simulink model "case30_governor"  (R2026a)
settings: Solver=ode14x  StopTime=8  FixedStep=0.001
values from neighbouring files (symbols this model uses):
  P = load('case30_simulink_data.mat')    [case30_build_model.m]    (also in case30_check_model.m = L.scenario_P(P0, B, Yr_pre, Vr_pre, TYPE, ALPHA, LOC, TF, TC; case30_compute_delta_p.m = P0; case30_compute_delta_p_small.m = P0; case30_generate_dataset.m = P0)
settings Model: Creator=rnoor  LastModifiedBy=rnoor

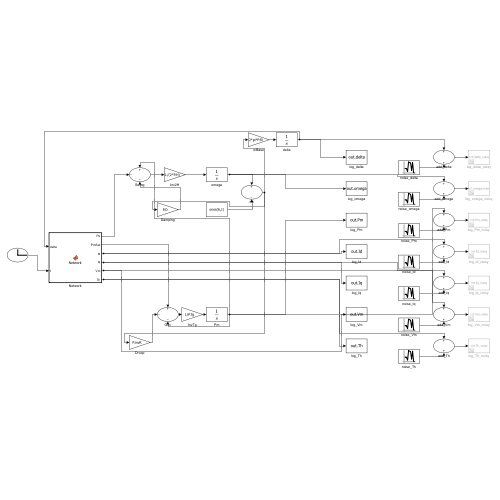
[thumbnail: Simulink's stored preview of the top-level diagram]
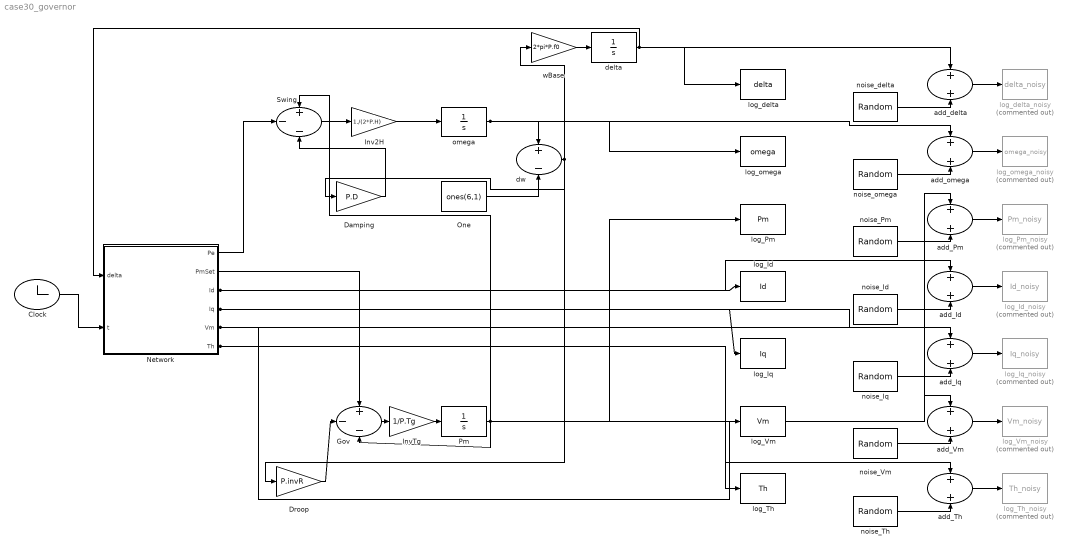
== system case30_governor ==
  Clock : Clock
  Damping : Gain  Gain=P.D
  Droop : Gain  Gain=P.invR
  Gov : Sum  Inputs=+--
  Inv2H : Gain  Gain=1./(2*P.H)
  InvTg : Gain  Gain=1/P.Tg
  Network : MATLAB Function  TreatAsAtomicUnit=on
  One : Constant  Value=ones(6,1)  VectorParams1D=off
  Pm : Integrator  InitialCondition=P.Pm0
  Swing : Sum  Inputs=+--
  add_Id : Sum
  add_Iq : Sum
  add_Pm : Sum
  add_Th : Sum
  add_Vm : Sum
  add_delta : Sum
  add_omega : Sum
  delta : Integrator  InitialCondition=P.delta0
  dw : Sum  Inputs=+-
  log_Id : ToWorkspace  VariableName=Id  SaveFormat=Timeseries  SampleTime=-1
  log_Id_noisy : ToWorkspace  Commented=on  VariableName=Id_noisy  SaveFormat=Timeseries  SampleTime=-1
  log_Iq : ToWorkspace  VariableName=Iq  SaveFormat=Timeseries  SampleTime=-1
  log_Iq_noisy : ToWorkspace  Commented=on  VariableName=Iq_noisy  SaveFormat=Timeseries  SampleTime=-1
  log_Pm : ToWorkspace  VariableName=Pm  SaveFormat=Timeseries  SampleTime=-1
  log_Pm_noisy : ToWorkspace  Commented=on  VariableName=Pm_noisy  SaveFormat=Timeseries  SampleTime=-1
  log_Th : ToWorkspace  VariableName=Th  SaveFormat=Timeseries  SampleTime=-1
  log_Th_noisy : ToWorkspace  Commented=on  VariableName=Th_noisy  SaveFormat=Timeseries  SampleTime=-1
  log_Vm : ToWorkspace  VariableName=Vm  SaveFormat=Timeseries  SampleTime=-1
  log_Vm_noisy : ToWorkspace  Commented=on  VariableName=Vm_noisy  SaveFormat=Timeseries  SampleTime=-1
  log_delta : ToWorkspace  VariableName=delta  SaveFormat=Timeseries  SampleTime=-1
  log_delta_noisy : ToWorkspace  Commented=on  VariableName=delta_noisy  SaveFormat=Timeseries  SampleTime=-1
  log_omega : ToWorkspace  VariableName=omega  SaveFormat=Timeseries  SampleTime=-1
  log_omega_noisy : ToWorkspace  Commented=on  VariableName=omega_noisy  SaveFormat=Timeseries  SampleTime=-1
  noise_Id : RandomNumber  Mean=zeros(6,1)  Variance=2.5e-05*ones(6,1)  Seed=400+(1:6)'  SampleTime=0.001  VectorParams1D=off
  noise_Iq : RandomNumber  Mean=zeros(6,1)  Variance=2.5e-05*ones(6,1)  Seed=500+(1:6)'  SampleTime=0.001  VectorParams1D=off
  noise_Pm : RandomNumber  Mean=zeros(6,1)  Variance=2.5e-05*ones(6,1)  Seed=300+(1:6)'  SampleTime=0.001  VectorParams1D=off
  noise_Th : RandomNumber  Mean=zeros(30,1)  Variance=0.0001*ones(30,1)  Seed=700+(1:30)'  SampleTime=0.001  VectorParams1D=off
  noise_Vm : RandomNumber  Mean=zeros(30,1)  Variance=1e-06*ones(30,1)  Seed=600+(1:30)'  SampleTime=0.001  VectorParams1D=off
  noise_delta : RandomNumber  Mean=zeros(6,1)  Variance=0.0001*ones(6,1)  Seed=100+(1:6)'  SampleTime=0.001  VectorParams1D=off
  noise_omega : RandomNumber  Mean=zeros(6,1)  Variance=2.5e-09*ones(6,1)  Seed=200+(1:6)'  SampleTime=0.001  VectorParams1D=off
  omega : Integrator  InitialCondition=ones(6,1)
  wBase : Gain  Gain=2*pi*P.f0
  wires:
  omega/1 -> dw/1, log_omega/1, add_omega/1
  One/1 -> dw/2
  dw/1 -> wBase/1, Damping/1, Droop/1
  wBase/1 -> delta/1
  Pm/1 -> Swing/1, Gov/3, log_Pm/1, add_Pm/1
  Network/1(Pe) -> Swing/2
  Damping/1 -> Swing/3
  Swing/1 -> Inv2H/1
  Inv2H/1 -> omega/1
  Network/2(PmSet) -> Gov/1
  Droop/1 -> Gov/2
  Gov/1 -> InvTg/1
  InvTg/1 -> Pm/1
  delta/1 -> Network/1(delta), log_delta/1, add_delta/1
  Clock/1 -> Network/2(t)
  noise_delta/1 -> add_delta/2
  add_delta/1 -> log_delta_noisy/1
  noise_omega/1 -> add_omega/2
  add_omega/1 -> log_omega_noisy/1
  noise_Pm/1 -> add_Pm/2
  add_Pm/1 -> log_Pm_noisy/1
  Network/3(Id) -> log_Id/1, add_Id/1
  noise_Id/1 -> add_Id/2
  add_Id/1 -> log_Id_noisy/1
  Network/4(Iq) -> log_Iq/1, add_Iq/1
  noise_Iq/1 -> add_Iq/2
  add_Iq/1 -> log_Iq_noisy/1
  Network/5(Vm) -> log_Vm/1, add_Vm/1
  noise_Vm/1 -> add_Vm/2
  add_Vm/1 -> log_Vm_noisy/1
  Network/6(Th) -> log_Th/1, add_Th/1
  noise_Th/1 -> add_Th/2
  add_Th/1 -> log_Th_noisy/1

== matlab function case30_governor/Network ==
  data: delta input; Pe output; t input; PmSet output; Id output; Iq output; Vm output; Th output; P parameter
function [Pe, PmSet, Id, Iq, Vm, Th] = Network(delta, t, P)
% Kron-reduced network; fault / clearing / delta_p switching by time
if t < P.t_fault - 1e-9
    Yr = P.Yred_pre;   Vr = P.Vrec_pre;   PmSet = P.Pm0;
elseif t < P.t_clear - 1e-9
    Yr = P.Yred_fault; Vr = P.Vrec_fault; PmSet = P.Pm0 + P.dPm0;
else
    Yr = P.Yred_post;  Vr = P.Vrec_post;  PmSet = P.Pm0;
end
if t >= P.t_corr - 1e-9 && t < P.t_corr_end - 1e-9
    PmSet = PmSet + P.dPc;               % corrective delta_p
end
rot = exp(1j*(delta(:) - pi/2));
E   = (P.Ed + 1j*P.Eq) .* rot;
I   = Yr * E;
Pe  = real(E .* conj(I));
Idq = I ./ rot;
Id  = real(Idq);  Iq = imag(Idq);
V   = Vr * E;
Vm  = abs(V);     Th = angle(V);
end
